simulink model "crs_controller_harness"  (R2026b)
settings: Solver=FixedStepDiscrete  FixedStep=Ts
settings Model: DataDictionary=crs_controllerdic.sldd  Creator=alexkim  LastModifiedBy=alexkim
settings DataIOCC: DSMLogging=off  ReturnWorkspaceOutputs=off  SaveOutput=off  SaveTime=off  SignalLogging=off
settings OptimizationCC: DefaultParameterBehavior=Inlined  EfficientFloat2IntCast=on  EfficientTunableParamExpr=on  LifeSpan=inf  PassReuseOutputArgsAs=Individual arguments
settings DebuggingCC: AlgebraicLoopMsg=error  ArtificialAlgebraicLoopMsg=error  AssertControl=DisableAll  BlockPriorityViolationMsg=error  BusObjectLabelMismatch=error  CheckMatrixSingularityMsg=error  InheritedTsInSrcMsg=error  IntegerOverflowMsg=error  IntegerSaturationMsg=error  ModelReferenceDataLoggingMessage=error  ModelReferenceIOMismatchMessage=error  NonBusSignalsTreatedAsBus=error  ParameterPrecisionLossMsg=error  ParameterTunabilityLossMsg=error  ParameterUnderflowMsg=error  ReadBeforeWriteMsg=EnableAllAsError  RootOutportRequireBusObject=error  SFExecutionAtInitializationDiag=error  SFInvalidInputDataAccessInChartInitDiag=error  SFSelfTransitionDiag=error  SFTemporalDelaySmallerThanSampleTimeDiag=error  SFTransitionActionBeforeConditionDiag=error  SFTransitionOutsideNaturalParentDiag=error  SFUndirectedBroadcastEventsDiag=error  SFUnreachableExecutionPathDiag=error  SFcnCompatibilityMsg=error  SaveWithDisabledLinksMsg=error  SaveWithParameterizedLinksMsg=error  SigSpecEnsureSampleTimeMsg=error  SignalInfNanChecking=error  SignalLabelMismatchMsg=error  SignalRangeChecking=warning  SolverPrmCheckMsg=error  StateNameClashWarn=warning  StrictBusMsg=ErrorOnBusTreatedAsVector  TasksWithSamePriorityMsg=error  UnconnectedInputMsg=error  UnconnectedLineMsg=error  UnconnectedOutputMsg=error  UnderSpecifiedDataTypeMsg=error  UniqueDataStoreMsg=error  UnknownTsInhSupMsg=error  UnnecessaryDatatypeConvMsg=warning  VariantConditionMismatch=error  VectorMatrixConversionMsg=error  WriteAfterReadMsg=EnableAllAsError  WriteAfterWriteMsg=EnableAllAsError
settings SFSimCC: CustomCodeUndefinedFunction=UseInterfaceOnly  EnableRuntimeRecursion=off  MATLABDynamicMemAlloc=off  SimUseLocalCustomCode=off
settings RTWCC: DLArmComputeVersion=19.05  Description=Embedded Coder  GenCodeOnly=on  GenerateReport=on  GenerateTraceInfo=on  GenerateTraceReport=on  GenerateTraceReportEml=on  GenerateTraceReportSf=on  GenerateTraceReportSl=on  IncludeHyperlinkInReport=on  LaunchReport=on  RTWUseLocalCustomCode=off  SystemTargetFile=ert.tlc  TemplateMakefile=ert_default_tmf
settings CodeAppCC: ForceParamTrailComments=on  IgnoreCustomStorageClasses=off  InsertBlockDesc=on  MATLABFcnDesc=on  MATLABSourceComments=on  OperatorAnnotations=on  ReqsInCode=on  SFDataObjDesc=on  SimulinkDataObjDesc=on  StateflowObjectComments=on
settings ERTTargetCC: CastingMode=Standards  DynamicArrayContainerType=coder::array  EnableSignedLeftShifts=off  EnableSignedRightShifts=off  GenerateSampleERTMain=on  IncludeMdlTerminateFcn=off  ParenthesesLevel=Standards  PreserveExpressionOrder=on  SupportNonFinite=off  SuppressErrorStatus=on  UtilityFuncGeneration=Shared location

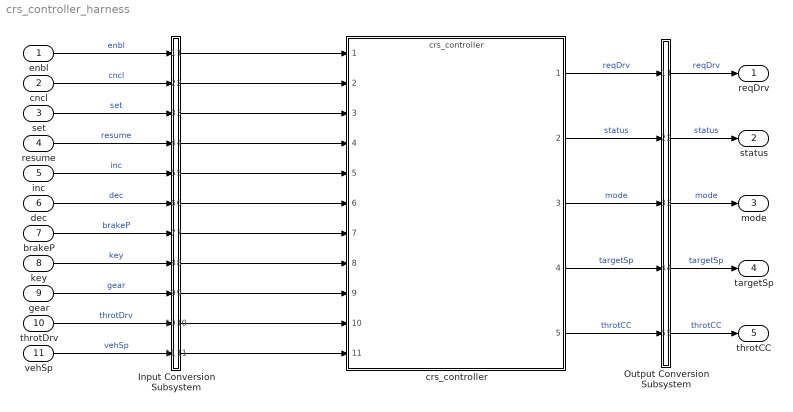
== system crs_controller_harness ==
  enbl : Inport  OutDataTypeStr=boolean  PortDimensions=[1]  SampleTime=0.01
  cncl : Inport  Port=2  OutDataTypeStr=boolean  PortDimensions=[1]  SampleTime=0.01
  set : Inport  Port=3  OutDataTypeStr=boolean  PortDimensions=[1]  SampleTime=0.01
  resume : Inport  Port=4  OutDataTypeStr=boolean  PortDimensions=[1]  SampleTime=0.01
  inc : Inport  Port=5  OutDataTypeStr=boolean  PortDimensions=[1]  SampleTime=0.01
  dec : Inport  Port=6  OutDataTypeStr=boolean  PortDimensions=[1]  SampleTime=0.01
  brakeP : Inport  Port=7  OutDataTypeStr=double  PortDimensions=[1]  SampleTime=0.01
  key : Inport  Port=8  OutDataTypeStr=uint8  PortDimensions=[1]  SampleTime=0.01
  gear : Inport  Port=9  OutDataTypeStr=uint8  PortDimensions=[1]  SampleTime=0.01
  throtDrv : Inport  Port=10  OutMin=0  OutMax=100  OutDataTypeStr=double  PortDimensions=[1]  SampleTime=0.01
  vehSp : Inport  Port=11  OutDataTypeStr=double  PortDimensions=[1]  SampleTime=0.01
  Input Conversion Subsystem : Subsystem  Tag=__SLT_ICS__  Description=|
      | Signal spec.
      | and routing
      settings: AttributesFormatString=%<Description>
  Output Conversion Subsystem : Subsystem  Tag=__SLT_OCS__  Description=|
      | Signal spec.
      | and routing
      settings: AttributesFormatString=%<Description>
  crs_controller : ModelReference  ModelNameDialog=crs_controller  SimulationMode=Normal  ModelReferenceVersion=16.2
  reqDrv : Outport
  status : Outport  Port=2
  mode : Outport  Port=3
  targetSp : Outport  Port=4
  throtCC : Outport  Port=5
  wires:
  enbl/1 -> Input Conversion Subsystem/1(Inport_1)  "enbl"
  cncl/1 -> Input Conversion Subsystem/2(Inport_2)  "cncl"
  set/1 -> Input Conversion Subsystem/3(Inport_3)  "set"
  resume/1 -> Input Conversion Subsystem/4(Inport_4)  "resume"
  inc/1 -> Input Conversion Subsystem/5(Inport_5)  "inc"
  dec/1 -> Input Conversion Subsystem/6(Inport_6)  "dec"
  brakeP/1 -> Input Conversion Subsystem/7(Inport_7)  "brakeP"
  key/1 -> Input Conversion Subsystem/8(Inport_8)  "key"
  gear/1 -> Input Conversion Subsystem/9(Inport_9)  "gear"
  throtDrv/1 -> Input Conversion Subsystem/10(Inport_10)  "throtDrv"
  vehSp/1 -> Input Conversion Subsystem/11(Inport_11)  "vehSp"
  Output Conversion Subsystem/1(Outport_1) -> reqDrv/1  "reqDrv"
  Output Conversion Subsystem/2(Outport_2) -> status/1  "status"
  Output Conversion Subsystem/3(Outport_3) -> mode/1  "mode"
  Output Conversion Subsystem/4(Outport_4) -> targetSp/1  "targetSp"
  Output Conversion Subsystem/5(Outport_5) -> throtCC/1  "throtCC"
  Input Conversion Subsystem/1(Outport_1) -> crs_controller/1
  Input Conversion Subsystem/2(Outport_2) -> crs_controller/2
  Input Conversion Subsystem/3(Outport_3) -> crs_controller/3
  Input Conversion Subsystem/4(Outport_4) -> crs_controller/4
  Input Conversion Subsystem/5(Outport_5) -> crs_controller/5
  Input Conversion Subsystem/6(Outport_6) -> crs_controller/6
  Input Conversion Subsystem/7(Outport_7) -> crs_controller/7
  Input Conversion Subsystem/8(Outport_8) -> crs_controller/8
  Input Conversion Subsystem/9(Outport_9) -> crs_controller/9
  Input Conversion Subsystem/10(Outport_10) -> crs_controller/10
  Input Conversion Subsystem/11(Outport_11) -> crs_controller/11
  crs_controller/1 -> Output Conversion Subsystem/1(Inport_1)  "reqDrv"
  crs_controller/2 -> Output Conversion Subsystem/2(Inport_2)  "status"
  crs_controller/3 -> Output Conversion Subsystem/3(Inport_3)  "mode"
  crs_controller/4 -> Output Conversion Subsystem/4(Inport_4)  "targetSp"
  crs_controller/5 -> Output Conversion Subsystem/5(Inport_5)  "throtCC"

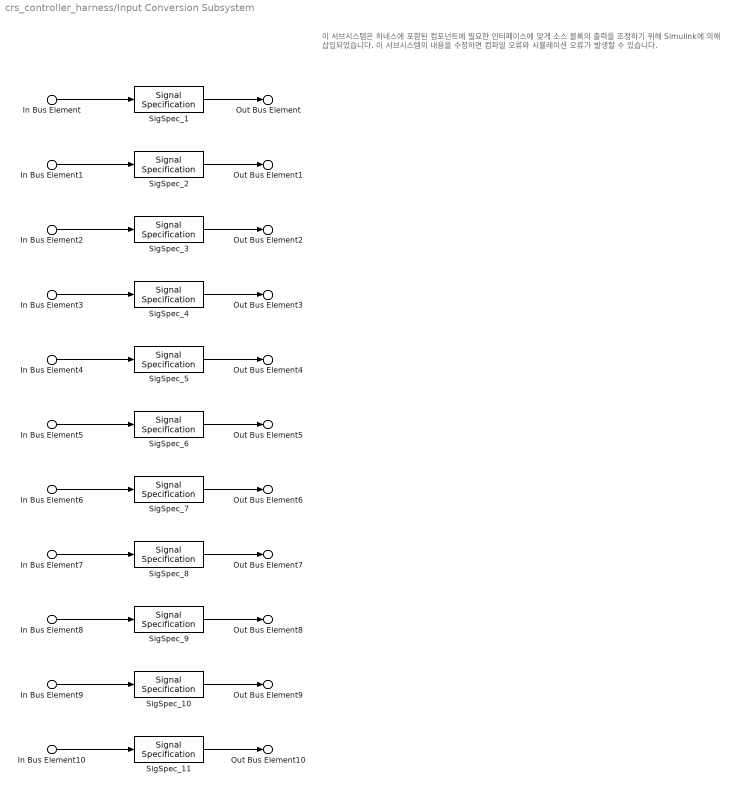
== system crs_controller_harness/Input Conversion Subsystem ==
  note: 이 서브시스템은 하네스에 포함된 컴포넌트에 필요한 인터페이스에 맞게 소스 블록의 출력을 조정하기 위해 Simulink에 의해 삽입되었습니다.
      |  이 서브시스템의 내용을 수정하면 컴파일 오류와 시뮬레이션 오류가 발생할 수 있습니다.
  In Bus Element : Inport  PortName=Inport_1
  In Bus Element1 : Inport  Port=2  PortName=Inport_2
  In Bus Element2 : Inport  Port=3  PortName=Inport_3
  In Bus Element3 : Inport  Port=4  PortName=Inport_4
  In Bus Element4 : Inport  Port=5  PortName=Inport_5
  In Bus Element5 : Inport  Port=6  PortName=Inport_6
  In Bus Element6 : Inport  Port=7  PortName=Inport_7
  In Bus Element7 : Inport  Port=8  PortName=Inport_8
  In Bus Element8 : Inport  Port=9  PortName=Inport_9
  In Bus Element9 : Inport  Port=10  PortName=Inport_10
  In Bus Element10 : Inport  Port=11  PortName=Inport_11
  SigSpec_{1..6} (6 alike) : SignalSpecification  OutDataTypeStr=boolean  Dimensions=[1]  SampleTime=0.01
  SigSpec_10 : SignalSpecification  OutDataTypeStr=double  Dimensions=[1]  SampleTime=0.01
  SigSpec_11 : SignalSpecification  OutDataTypeStr=double  Dimensions=[1]  SampleTime=0.01
  SigSpec_7 : SignalSpecification  OutDataTypeStr=double  Dimensions=[1]  SampleTime=0.01
  SigSpec_8 : SignalSpecification  OutDataTypeStr=uint8  Dimensions=[1]  SampleTime=0.01
  SigSpec_9 : SignalSpecification  OutDataTypeStr=uint8  Dimensions=[1]  SampleTime=0.01
  Out Bus Element : Outport  PortName=Outport_1
  Out Bus Element1 : Outport  Port=2  PortName=Outport_2
  Out Bus Element2 : Outport  Port=3  PortName=Outport_3
  Out Bus Element3 : Outport  Port=4  PortName=Outport_4
  Out Bus Element4 : Outport  Port=5  PortName=Outport_5
  Out Bus Element5 : Outport  Port=6  PortName=Outport_6
  Out Bus Element6 : Outport  Port=7  PortName=Outport_7
  Out Bus Element7 : Outport  Port=8  PortName=Outport_8
  Out Bus Element8 : Outport  Port=9  PortName=Outport_9
  Out Bus Element9 : Outport  Port=10  PortName=Outport_10
  Out Bus Element10 : Outport  Port=11  PortName=Outport_11
  wires:
  SigSpec_1/1 -> Out Bus Element/1
  In Bus Element/1 -> SigSpec_1/1
  SigSpec_2/1 -> Out Bus Element1/1
  In Bus Element1/1 -> SigSpec_2/1
  SigSpec_3/1 -> Out Bus Element2/1
  In Bus Element2/1 -> SigSpec_3/1
  SigSpec_4/1 -> Out Bus Element3/1
  In Bus Element3/1 -> SigSpec_4/1
  SigSpec_5/1 -> Out Bus Element4/1
  In Bus Element4/1 -> SigSpec_5/1
  SigSpec_6/1 -> Out Bus Element5/1
  In Bus Element5/1 -> SigSpec_6/1
  SigSpec_7/1 -> Out Bus Element6/1
  In Bus Element6/1 -> SigSpec_7/1
  SigSpec_8/1 -> Out Bus Element7/1
  In Bus Element7/1 -> SigSpec_8/1
  SigSpec_9/1 -> Out Bus Element8/1
  In Bus Element8/1 -> SigSpec_9/1
  SigSpec_10/1 -> Out Bus Element9/1
  In Bus Element9/1 -> SigSpec_10/1
  SigSpec_11/1 -> Out Bus Element10/1
  In Bus Element10/1 -> SigSpec_11/1

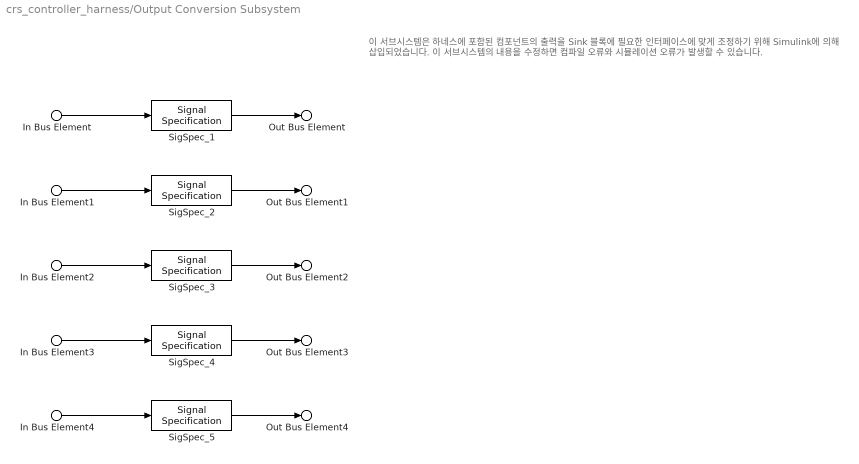
== system crs_controller_harness/Output Conversion Subsystem ==
  note: 이 서브시스템은 하네스에 포함된 컴포넌트의 출력을 Sink 블록에 필요한 인터페이스에 맞게 조정하기 위해 Simulink에 의해 삽입되었습니다.
      |  이 서브시스템의 내용을 수정하면 컴파일 오류와 시뮬레이션 오류가 발생할 수 있습니다.
  In Bus Element : Inport  PortName=Inport_1
  In Bus Element1 : Inport  Port=2  PortName=Inport_2
  In Bus Element2 : Inport  Port=3  PortName=Inport_3
  In Bus Element3 : Inport  Port=4  PortName=Inport_4
  In Bus Element4 : Inport  Port=5  PortName=Inport_5
  SigSpec_1 : SignalSpecification  OutDataTypeStr=Enum: reqMode  Dimensions=[1]  SampleTime=0.01
  SigSpec_2 : SignalSpecification  OutDataTypeStr=boolean  Dimensions=[1]  SampleTime=0.01
  SigSpec_3 : SignalSpecification  OutDataTypeStr=Enum: opMode  Dimensions=[1]  SampleTime=0.01
  SigSpec_4 : SignalSpecification  OutDataTypeStr=double  Dimensions=[1]  SampleTime=0.01
  SigSpec_5 : SignalSpecification  OutDataTypeStr=double  Dimensions=[1]  SampleTime=0.01
  Out Bus Element : Outport  PortName=Outport_1
  Out Bus Element1 : Outport  Port=2  PortName=Outport_2
  Out Bus Element2 : Outport  Port=3  PortName=Outport_3
  Out Bus Element3 : Outport  Port=4  PortName=Outport_4
  Out Bus Element4 : Outport  Port=5  PortName=Outport_5
  wires:
  In Bus Element/1 -> SigSpec_1/1
  SigSpec_1/1 -> Out Bus Element/1
  In Bus Element1/1 -> SigSpec_2/1
  SigSpec_2/1 -> Out Bus Element1/1
  In Bus Element2/1 -> SigSpec_3/1
  SigSpec_3/1 -> Out Bus Element2/1
  In Bus Element3/1 -> SigSpec_4/1
  SigSpec_4/1 -> Out Bus Element3/1
  In Bus Element4/1 -> SigSpec_5/1
  SigSpec_5/1 -> Out Bus Element4/1
